simulink model "pid_aw_ctrl"  (R2025b)
settings: Solver=FixedStepDiscrete  StartTime=0.0  StopTime=10.0  FixedStep=Ts  RelTol=1e-3
PreLoadFcn:
  | Ts = 1e-3; tau = 0.01; ad = exp(-Ts/tau); bd = 1 - ad;
undefined symbols (not defined in the file or in its folder): pid_aw_init
settings Model: Creator=jnune  LastModifiedBy=jnune
settings OptimizationCC: DefaultParameterBehavior=Inlined  EnhancedBackFolding=on  PassReuseOutputArgsAs=Individual arguments  ZeroExternalMemoryAtStartup=off  ZeroInternalMemoryAtStartup=off  MaxStackSize=64  OptimizeBlockOrder=speed  DifferentSizesBufferReuse=on  OptimizationCustomize=off  EfficientTunableParamExpr=on
settings DebuggingCC: ParameterPrecisionLossMsg=none  ParameterTunabilityLossMsg=error
settings HardwareCC: ProdBitPerPointer=32.0  ProdBitPerSizeT=32.0  ProdBitPerPtrDiffT=32.0  ProdLargestAtomicInteger=Long  ProdLargestAtomicFloat=Double  ProdWordSize=32.0  ProdLongLongMode=on  ProdHWDeviceType=ARM Compatible->ARM Cortex-M
settings ModelReferenceCC: ModelReferenceNumInstancesAllowed=Single  SupportModelReferenceSimTargetCustomCode=on
settings SFSimCC: SimCustomHeaderCode="#include \"pid_aw.h\""  SimUserSources=C:\Escritorio\Memoria\PID_PIL_C\pid_aw.c  SimUserIncludeDirs=C:\Escritorio\Memoria\PID_PIL_C  MATLABDynamicMemAlloc=off
settings RTWCC: SystemTargetFile=ert.tlc  HardwareBoard=STM32 Nucleo F767ZI  TemplateMakefile=ert_default_tmf  CustomHeaderCode="#include \"pid_aw.h\""  CustomInclude=C:\Escritorio\Memoria\PID_PIL_C  CustomSource=C:\Escritorio\Memoria\PID_PIL_C\pid_aw.c  Toolchain=GNU Tools for ARM Embedded Processors  Description=Embedded Coder
settings CodeAppCC: ForceParamTrailComments=on  IgnoreCustomStorageClasses=off  OperatorAnnotations=on  SimulinkDataObjDesc=on  SFDataObjDesc=on  InsertBlockDesc=on
settings ERTTargetCC: ExtModeTransport=3.0  ExtModeStaticAlloc=on  ExtModeStaticAllocSize=2000.0  ExtModeMexFile=ext_xcp  ExtModeIntrfLevel=Level2 - Open  TargetLangStandard=C99 (ISO)  SubcomponentCodeInterfacePackaging=Nonreusable function

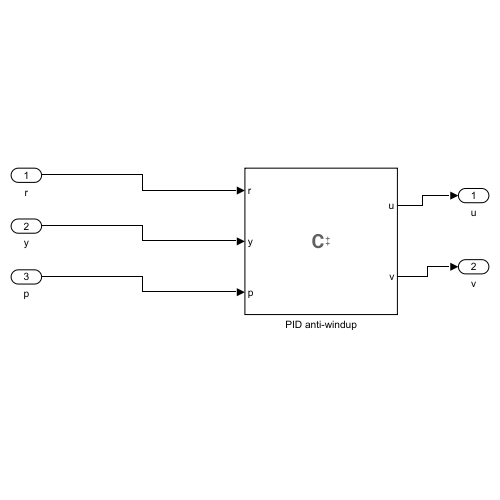
[thumbnail: Simulink's stored preview of the top-level diagram]
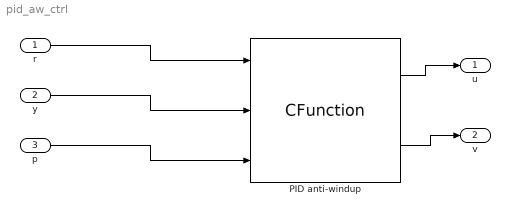
== system pid_aw_ctrl ==
  r : Inport  SampleTime=Ts
  y : Inport  Port=2  SampleTime=Ts
  p : Inport  Port=3  PortDimensions=8  SampleTime=Ts
  PID anti-windup : CFunction  OutputCode=|  StartCode=pid_aw_init();  CodegenOutputCode=|  CodegenStartCode=pid_aw_init();  SampleTime=Ts  CustomCodeSettingLocation=ModelConfigurationParameters
      OutputCode=|
      | double vv;
      | u = pid_aw_step(r, y, p, &vv);
      | v = vv;
      CodegenOutputCode=|
      | double vv;
      | u = pid_aw_step(r, y, p, &vv);
      | v = vv;
  u : Outport
  v : Outport  Port=2
  wires:
  r/1 -> PID anti-windup/1
  y/1 -> PID anti-windup/2
  p/1 -> PID anti-windup/3
  PID anti-windup/1 -> u/1
  PID anti-windup/2 -> v/1
